simulink library "indi_lib"  (R2018b)
settings: Solver=VariableStepAuto  StartTime=0.0  StopTime=10.0  RelTol=1e-3
values from neighbouring files (symbols this model uses):
  G10 = [          inv_I_b * cross( pos, c_XYZ );          c_XYZ / ceb.m      ]    [indiCeFlapFix.m]    (also in indiCePropFix.m = [          2 * inv_I_b * (cep.k*L + cep.d*M .* repmat(cep.a,)
  G20 = 1 / T_s *      [          inv_I_b * cep.ip * M .* repmat(cep.a,3,1);          zeros( 1, num_motors )      ]    [indiCePropFix.m]
undefined symbols (not defined in the file or in its folder): ap, ca, ceb, cep, indiCePropAffineCntrl, lindi, mtc, sflt, sflt_omega, ts
libraries: filters_lib x6, $bdroot x2, ca_lib x2, ndi_lib x2, simulink x1
settings Model: Creator=Ybeyer  LastModifiedBy=jonas
settings DebuggingCC: LibraryContextMissingDiagnostic=none
settings SFSimCC: SimUseLocalCustomCode=off
settings RTWCC: RTWUseLocalCustomCode=off
settings CodeAppCC: StateflowObjectComments=on

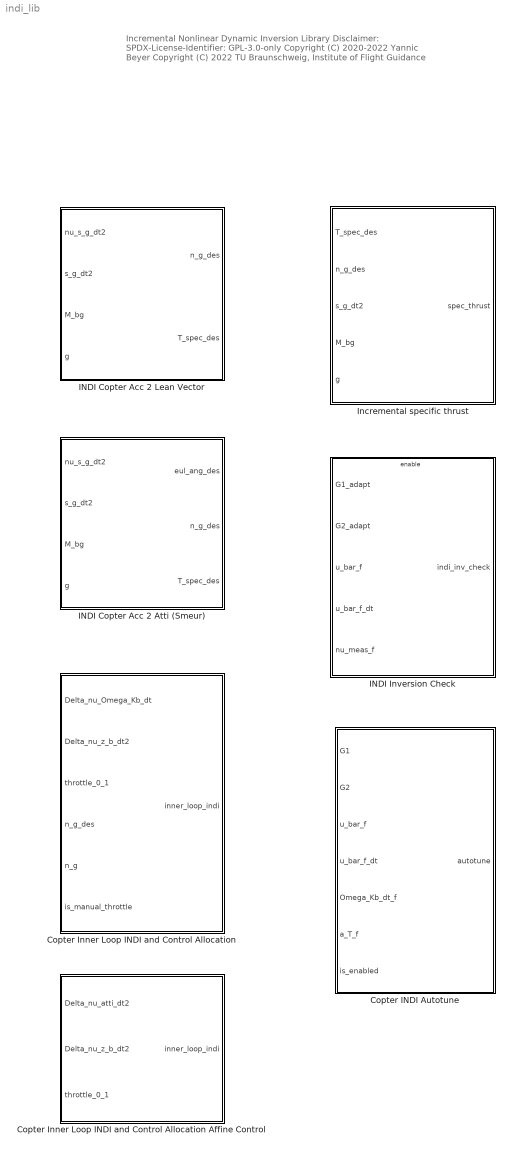
== system indi_lib ==
  note: Incremental Nonlinear Dynamic Inversion Library
      |
      | Disclaimer:
      | SPDX-License-Identifier: GPL-3.0-only
      |
      | Copyright (C) 2020-2022 Yannic Beyer
      | Copyright (C) 2022 TU Braunschweig, Institute of Flight Guidance
  Copter INDI Autotune : Subsystem  mask{rm_atc=lindi.atc.rm, mtc=lindi.mtc, sflt_omega=lindi.sflt.omega, ts=lindi.ts}
      mask prompts: rm_atc "Attitude reference model parameters struct"; mtc "Motor time constant, s"; sflt_omega "Sensor filter cutoff frequency, rad/s"; ts "Sample time, s"
      mask DialogControl DescGroupVar Prompt: Copter INDI Autotune
      mask DialogControl DescTextVar Prompt: This adaptive INDI block is based on: Smeur, E. J., Chu, Q., & De Croon, G. C. (2016). Adaptive incremental nonlinear dynamic inversion for attitude control of micro air vehicles. Journal of Guidance, Control, and Dynamics, 39(3), 450-461.
      mask DialogControl Control2 Prompt: Instead of finding all entries in the G1 and G2 matrix, the number of estimated parameters is 5: one for each: roll, pitch, yaw, vertical acc. (G1) and one for yaw due to propeller acceleration (G2).
  Copter Inner Loop INDI and Control Allocation : Subsystem  mask{cep=ap.cep, ceb=ap.ceb, ca=ap.ca, mtc=ap.mtc, sflt=ap.sflt, ts=ap.ts, is_ce_extern=off}
      mask prompts: cep "Parameters for motor-propeller control effectiveness, see indiCeProp_params_default"; ceb "Parameters for body control effectiveness, see indiCeBody_params_default"; ca "Control allocation parameters, see controlAllocationWlsLoadParams"; mtc "Motor time constant, s"; sflt "Sensor filter parameters, see indiSensFiltLoadParams"; ts "Sample time, s"; is_ce_extern "Enable external control effectiveness"
      mask init:
      | caIndiCopterBlockInit(is_ce_extern);
      mask DialogControl DescGroupVar Prompt: Copter Inner Loop INDI and Control Allocation
  Copter Inner Loop INDI and Control Allocation Affine Control : Subsystem  mask{cep=cep, ceb=ceb, ca=ca, mtc=mtc, sflt=sflt, ts=ts}
      mask prompts: cep "Parameters for motor-propeller control effectiveness, see indiCeProp_params_default"; ceb "Parameters for body control effectiveness, see indiCeBody_params_default"; ca "Control allocation parameters, see controlAllocationWlsLoadParams"; mtc "Motor time constant, s"; sflt "Sensor filter parameters, see indiSensFiltLoadParams"; ts "Sample time, s"
      mask init:
      | u_min = ca.u_min;
      | u_max = ca.u_max;
      | u_d = ca.u_d;
      | 
      | U_min = indiCePropAffineCntrl( cep, ca.u_min );
      | U_max = indiCePropAffineCntrl( cep, ca.u_max );
      | U_d = indiCePropAffineCntrl( cep, ca.u_d );
      | 
      | ca.u_min = U_min;
      | ca.u_max = U_max;
      | ca.u_d = U_d;
      mask DialogControl DescGroupVar Prompt: Copter Inner Loop INDI and Control Allocation with Affine Control
      mask DialogControl DescTextVar Prompt: The special feature of this implementation is that the control effectiveness matrix G1 (or renamed G1U here) remains constant, so it does not need to be scheduled. For this purpose, an artificial control input (here called 0 <= U <= 1) was defined, on which the thrust and the torque depend linearly. The actual control input (duty cycle 0 <= u <= 1) is then calculated non-linearly from the artificial control input U.
  INDI Copter Acc 2 Atti (Smeur) : MATLAB Function  TreatAsAtomicUnit=on
  INDI Copter Acc 2 Lean Vector : MATLAB Function  TreatAsAtomicUnit=on
  INDI Inversion Check : Subsystem  mask{omega_filt=2/(2/sflt_omega + mtc), mask_expr_handling_config=default}
      mask prompts: omega_filt "Filter cutoff frequency (sensor and actuator), rad/s"
      mask init:
      | maskExprHandling(gcbh, mask_expr_handling_config);
      mask TypeOptions mask_expr_handling_config: default | passthrough (tunable)
      mask DialogControl DescGroupVar Prompt: INDI Inversion Check
      mask DialogControl DescTextVar Prompt: Check how good an INDI inversion is. Therefore, the expected and measure pseudo-control signal can be compared.
      mask DialogControl CodeGenerationSettings Prompt: Code Generation Settings
      mask DialogControl maskExprHandlingText Prompt: Mask expression handling
      mask DialogControl maskExprHandlingReadme Prompt: README
      mask DialogControl maskExprHandlingReadme Tooltip: https://github.com/iff-gsc/m-Utils/tree/main/simulink/mask_expression_handling/README.md
      mask DialogControl maskExprHandlingReadme Callback: web('https://github.com/iff-gsc/m-Utils/tree/main/simulink/mask_expression_handling/README.md','-browser')
  Incremental specific thrust : Subsystem  mask{leanfreq=10, leandamp=1, is_enable_checked=off, states_when_enabling=held}
      mask prompts: leanfreq "Natural frequency of attitude reference model, rad/s"; leandamp "Damping ratio of attitude reference model"; is_enable_checked "Activate "Enabled Subsystem""; states_when_enabling "States when enabling:"
      mask init:
      | cntrlBlockInit(is_enable_checked,states_when_enabling);
      mask TypeOptions states_when_enabling: held | reset
      mask DialogControl DescGroupVar Prompt: Incremental specific thrust

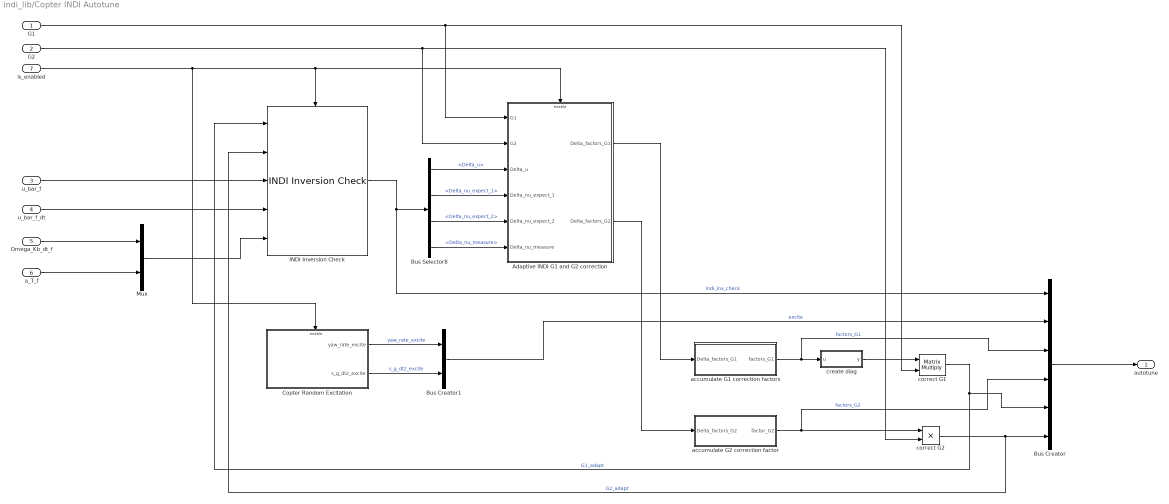
== system indi_lib/Copter INDI Autotune ==
  G1 : Inport
  G2 : Inport  Port=2
  u_bar_f : Inport  Port=3
  u_bar_f_dt : Inport  Port=4
  Omega_Kb_dt_f : Inport  Port=5
  a_T_f : Inport  Port=6
  is_enabled : Inport  Port=7
  Adaptive INDI G1 and G2 correction : Subsystem
  Bus Creator : BusCreator  Inputs=6
  Bus Creator1 : BusCreator  Inputs=2
  Bus Selector8 : BusSelector  OutputSignals=Delta_u,Delta_nu_expect_1,Delta_nu_expect_2,Delta_nu_measure
  Copter Random Excitation : Subsystem
  INDI Inversion Check : $bdroot/INDI Inversion Check  omega_filt=2/(2/sflt_omega + mtc)  mask_expr_handling_config=passthrough (tunable)
  Mux : Mux  Inputs=2
  accumulate G1 correction factors : Subsystem
  accumulate G2 correction factor : Subsystem
  correct G1 : Product  Multiplication=Matrix(*)
  correct G2 : Product
  create diag : MATLAB Function  TreatAsAtomicUnit=on
  autotune : Outport
  wires:
  G1/1 -> Adaptive INDI G1 and G2 correction/1(G1), correct G1/2
  G2/1 -> correct G2/2, Adaptive INDI G1 and G2 correction/2(G2)
  Adaptive INDI G1 and G2 correction/1(Delta_factors_G1) -> accumulate G1 correction factors/1(Delta_factors_G1)
  accumulate G1 correction factors/1(factors_G1) -> Bus Creator/3, create diag/1(u)  "factors_G1"
  accumulate G2 correction factor/1(factor_G2) -> Bus Creator/4, correct G2/1  "factors_G2"
  Adaptive INDI G1 and G2 correction/2(Delta_factors_G2) -> accumulate G2 correction factor/1(Delta_factors_G2)
  Copter Random Excitation/2(s_g_dt2_excite) -> Bus Creator1/2  "s_g_dt2_excite"
  Bus Selector8/2 -> Adaptive INDI G1 and G2 correction/4(Delta_nu_expect_1)  "<Delta_nu_expect_1>"
  Copter Random Excitation/1(yaw_rate_excite) -> Bus Creator1/1  "yaw_rate_excite"
  Bus Selector8/1 -> Adaptive INDI G1 and G2 correction/3(Delta_u)  "<Delta_u>"
  Bus Selector8/3 -> Adaptive INDI G1 and G2 correction/5(Delta_nu_expect_2)  "<Delta_nu_expect_2>"
  INDI Inversion Check/1 -> Bus Creator/1, Bus Selector8/1  "indi_inv_check"
  Bus Selector8/4 -> Adaptive INDI G1 and G2 correction/6(Delta_nu_measure)  "<Delta_nu_measure>"
  Bus Creator1/1 -> Bus Creator/2  "excite"
  Bus Creator/1 -> autotune/1
  Mux/1 -> INDI Inversion Check/5
  u_bar_f/1 -> INDI Inversion Check/3
  u_bar_f_dt/1 -> INDI Inversion Check/4
  Omega_Kb_dt_f/1 -> Mux/1
  a_T_f/1 -> Mux/2
  correct G2/1 -> Bus Creator/6, INDI Inversion Check/2  "G2_adapt"
  correct G1/1 -> INDI Inversion Check/1, Bus Creator/5  "G1_adapt"
  create diag/1(y) -> correct G1/1
  is_enabled/1 -> INDI Inversion Check/Enable, Adaptive INDI G1 and G2 correction/Enable, Copter Random Excitation/Enable

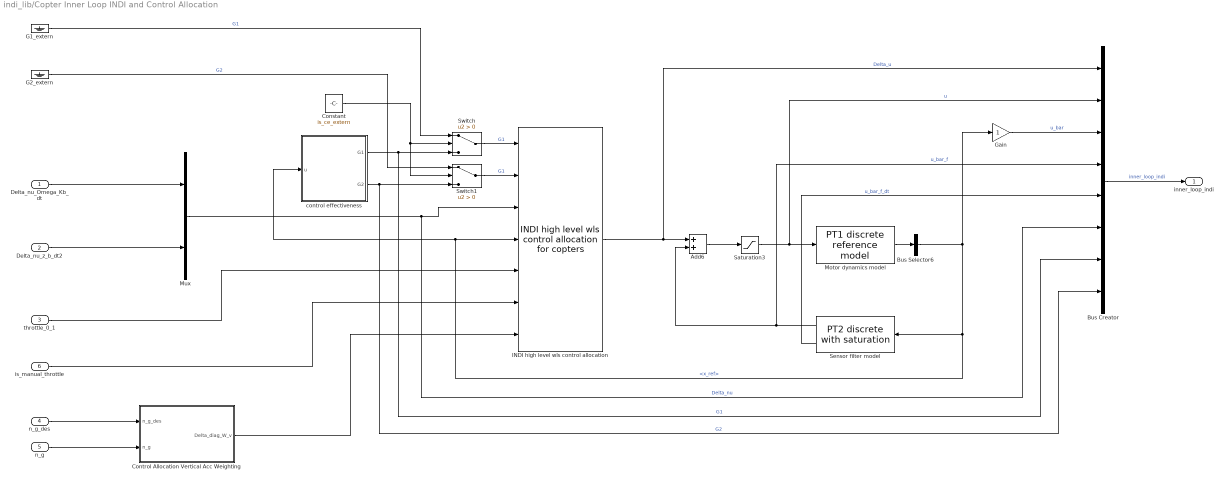
== system indi_lib/Copter Inner Loop INDI and Control Allocation ==
  Delta_nu_Omega_Kb_dt : Inport
  Delta_nu_z_b_dt2 : Inport  Port=2
  throttle_0_1 : Inport  Port=3
  n_g_des : Inport  Port=4
  n_g : Inport  Port=5
  is_manual_throttle : Inport  Port=6
  Add6 : Sum
  Bus Creator : BusCreator  Inputs=8
  Bus Selector6 : BusSelector  OutputSignals=x_ref
  Constant : Constant  Value=is_ce_extern
  Control Allocation Vertical Acc Weighting : MATLAB Function  TreatAsAtomicUnit=on
  G1_extern : Ground
  G2_extern : Ground
  Gain : Gain
  INDI high level wls control allocation : ca_lib/INDI high level wls control allocation for copters  ca=ca  is_Delta_W_v_check=on  is_W_check=off  is_iter_check=off
      settings: SourceProductName=LADAC
  Motor dynamics model : ndi_lib/PT1 discrete reference model  T=mtc  x_max=inf  x_min=-inf  x_dt_max=inf  x_dt_min=-inf  x_init=0
      settings: SourceProductName=LADAC
  Mux : Mux  Inputs=2
  Saturation3 : Saturate  UpperLimit=ca.u_max  LowerLimit=ca.u_min
  Sensor filter model : filters_lib/PT2 discrete with saturation  param_src=internal  omega=sflt.omega  d=sflt.D  x_max=inf  x_min=-inf  x_dt_max=inf  x_dt_min=-inf  x_dt2_max=inf  x_dt2_min=-inf  y_0_src=internal  x_init=0  y_dt_0_src=internal  x_dt_init=0  is_y_dt_checked=on  is_y_dt2_checked=off  is_external_reset_checked=off  mask_expr_handling_config=default
      settings: SourceProductName=LADAC
  Switch : Switch  Criteria=u2 > Threshold
  Switch1 : Switch  Criteria=u2 > Threshold
  control effectiveness : Subsystem  mask{cep=cep, ceb=ceb, ts=ts, u_min=ca.u_min}
      mask prompts: cep "propeller control effectiveness struct, see cntrlEffectPropLoadParams"; ceb "body control effectiveness struct, see cntrlEffectBodyLoadParams"; ts "controller sample time, s"
      mask init:
      | [G10,G20] = indiCePropFix( cep, ceb, ts );
  inner_loop_indi : Outport
  wires:
  is_manual_throttle/1 -> INDI high level wls control allocation/6
  n_g/1 -> Control Allocation Vertical Acc Weighting/2(n_g)
  n_g_des/1 -> Control Allocation Vertical Acc Weighting/1(n_g_des)
  Control Allocation Vertical Acc Weighting/1(Delta_diag_W_v) -> INDI high level wls control allocation/7
  Bus Creator/1 -> inner_loop_indi/1  "inner_loop_indi"
  Gain/1 -> Bus Creator/3  "u_bar"
  Delta_nu_z_b_dt2/1 -> Mux/2
  control effectiveness/2(G2) -> Switch1/3, Bus Creator/8  "G2"
  Delta_nu_Omega_Kb_dt/1 -> Mux/1
  Add6/1 -> Saturation3/1
  Motor dynamics model/1 -> Bus Selector6/1
  control effectiveness/1(G1) -> Bus Creator/7, Switch/3  "G1"
  Bus Selector6/1 -> control effectiveness/1(u), INDI high level wls control allocation/4, Sensor filter model/1, Gain/1  "<x_ref>"
  throttle_0_1/1 -> INDI high level wls control allocation/5
  INDI high level wls control allocation/1 -> Add6/1, Bus Creator/1  "Delta_u"
  Saturation3/1 -> Motor dynamics model/1, Bus Creator/2  "u"
  Mux/1 -> Bus Creator/6, INDI high level wls control allocation/3  "Delta_nu"
  Sensor filter model/1 -> Add6/2, Bus Creator/4  "u_bar_f"
  Switch/1 -> INDI high level wls control allocation/1  "G1"
  Switch1/1 -> INDI high level wls control allocation/2  "G1"
  G1_extern/1 -> Switch/1  "G1"
  G2_extern/1 -> Switch1/1  "G2"
  Constant/1 -> Switch1/2, Switch/2
  Sensor filter model/2 -> Bus Creator/5  "u_bar_f_dt"

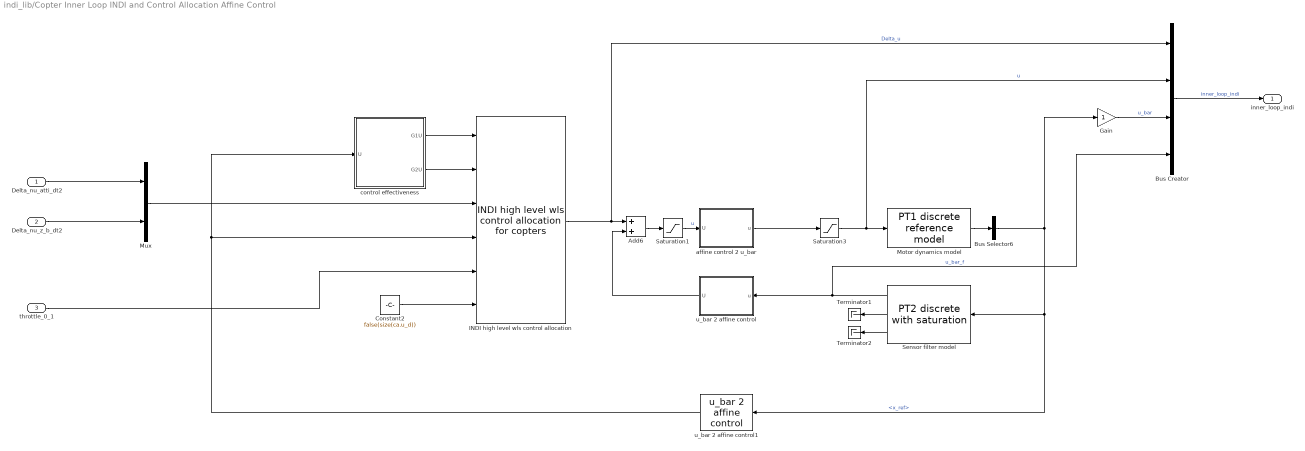
== system indi_lib/Copter Inner Loop INDI and Control Allocation Affine Control ==
  Delta_nu_atti_dt2 : Inport
  Delta_nu_z_b_dt2 : Inport  Port=2
  throttle_0_1 : Inport  Port=3
  Add6 : Sum
  Bus Creator : BusCreator  Inputs=4
  Bus Selector6 : BusSelector  OutputSignals=x_ref
  Constant2 : Constant  Value=false(size(ca.u_d))
  Gain : Gain
  INDI high level wls control allocation : ca_lib/INDI high level wls control allocation for copters  ca=ca  is_Delta_W_v_check=off  is_W_check=off  is_iter_check=off
      settings: SourceProductName=LADAC
  Motor dynamics model : ndi_lib/PT1 discrete reference model  T=mtc  x_max=inf  x_min=-inf  x_dt_max=inf  x_dt_min=-inf  x_init=0
      settings: SourceProductName=LADAC
  Mux : Mux  Inputs=2
  Saturation1 : Saturate  UpperLimit=indiCePropAffineCntrl( cep, ca.u_max )  LowerLimit=indiCePropAffineCntrl( cep, ca.u_min )
  Saturation3 : Saturate  UpperLimit=u_max  LowerLimit=u_min
  Sensor filter model : filters_lib/PT2 discrete with saturation  param_src=internal  omega=sflt.omega  d=sflt.D  x_dt2_max=inf  x_dt2_min=-inf  x_dt_max=inf  x_dt_min=-inf  x_max=inf  x_min=-inf  y_0_src=internal  x_init=0  y_dt_0_src=internal  x_dt_init=0  is_y_dt_checked=on  is_y_dt2_checked=on
      settings: SourceProductName=LADAC
  Terminator1 : Terminator
  Terminator2 : Terminator
  affine control 2 u_bar : Subsystem  mask{cep=cep}
  control effectiveness : Subsystem  mask{cep=cep, ceb=ceb, ts=ts, u_min=ca.u_min}
      mask prompts: cep "propeller control effectiveness struct, see cntrlEffectPropLoadParams"; ceb "body control effectiveness struct, see cntrlEffectBodyLoadParams"; ts "controller sample time, s"
      mask init:
      | [G10,G20] = indiCePropFix( cep, ceb, ts );
      | 
      | u_max = ones(4,1);
      | 
      | omega_max = motorStaticSpeed( cep.kt, cep.ri, cep.vb, cep.d, u_max );
      | omega2 = diag( omega_max.^2 );
      | 
      | G1U = 0.5 * G10 * omega2;
  u_bar 2 affine control : Subsystem  mask{cep=cep}
  u_bar 2 affine control1 : $bdroot/Copter Inner Loop INDI and Control Allocation Affine Control/u_bar 2 affine control  cep=cep
  inner_loop_indi : Outport
  wires:
  throttle_0_1/1 -> INDI high level wls control allocation/5
  Sensor filter model/1 -> Bus Creator/4, u_bar 2 affine control/1(u)  "u_bar_f"
  Sensor filter model/2 -> Terminator1/1
  Add6/1 -> Saturation1/1
  INDI high level wls control allocation/1 -> Bus Creator/1, Add6/1  "Delta_u"
  affine control 2 u_bar/1(u) -> Saturation3/1
  Motor dynamics model/1 -> Bus Selector6/1
  Constant2/1 -> INDI high level wls control allocation/6
  Sensor filter model/3 -> Terminator2/1
  Delta_nu_atti_dt2/1 -> Mux/1
  Saturation3/1 -> Bus Creator/2, Motor dynamics model/1  "u"
  u_bar 2 affine control1/1 -> control effectiveness/1(U), INDI high level wls control allocation/4
  Bus Selector6/1 -> Gain/1, u_bar 2 affine control1/1, Sensor filter model/1  "<x_ref>"
  Delta_nu_z_b_dt2/1 -> Mux/2
  Saturation1/1 -> affine control 2 u_bar/1(U)  "u"
  Mux/1 -> INDI high level wls control allocation/3
  u_bar 2 affine control/1(U) -> Add6/2
  control effectiveness/1(G1U) -> INDI high level wls control allocation/1
  control effectiveness/2(G2U) -> INDI high level wls control allocation/2
  Bus Creator/1 -> inner_loop_indi/1  "inner_loop_indi"
  Gain/1 -> Bus Creator/3  "u_bar"

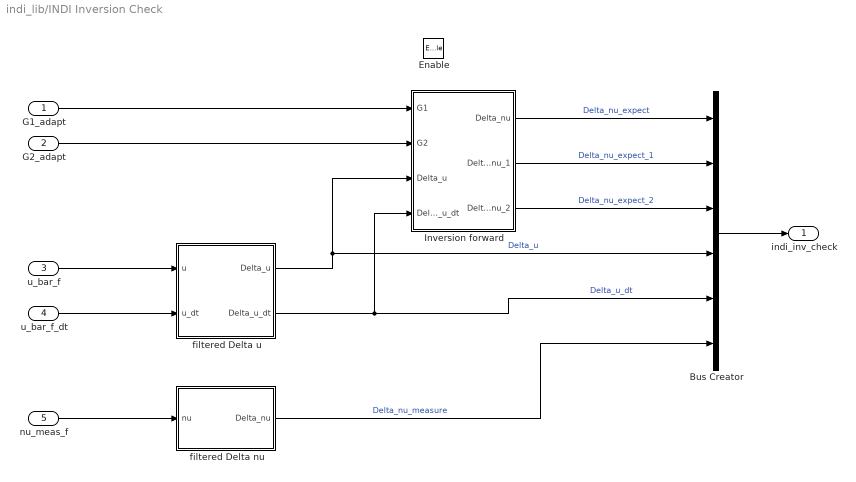
== system indi_lib/INDI Inversion Check ==
  G1_adapt : Inport
  G2_adapt : Inport  Port=2
  u_bar_f : Inport  Port=3
  u_bar_f_dt : Inport  Port=4
  nu_meas_f : Inport  Port=5
  Enable : EnablePort
  Bus Creator : BusCreator  Inputs=6
  Inversion forward : Subsystem
  filtered Delta nu : Subsystem
  filtered Delta u : Subsystem
  indi_inv_check : Outport
  wires:
  Inversion forward/3(Delta_nu_2) -> Bus Creator/3  "Delta_nu_expect_2"
  Inversion forward/2(Delta_nu_1) -> Bus Creator/2  "Delta_nu_expect_1"
  G1_adapt/1 -> Inversion forward/1(G1)
  G2_adapt/1 -> Inversion forward/2(G2)
  Inversion forward/1(Delta_nu) -> Bus Creator/1  "Delta_nu_expect"
  u_bar_f/1 -> filtered Delta u/1(u)
  filtered Delta u/1(Delta_u) -> Inversion forward/3(Delta_u), Bus Creator/4  "Delta_u"
  filtered Delta nu/1(Delta_nu) -> Bus Creator/6  "Delta_nu_measure"
  nu_meas_f/1 -> filtered Delta nu/1(nu)
  u_bar_f_dt/1 -> filtered Delta u/2(u_dt)
  filtered Delta u/2(Delta_u_dt) -> Bus Creator/5, Inversion forward/4(Delta_u_dt)  "Delta_u_dt"
  Bus Creator/1 -> indi_inv_check/1

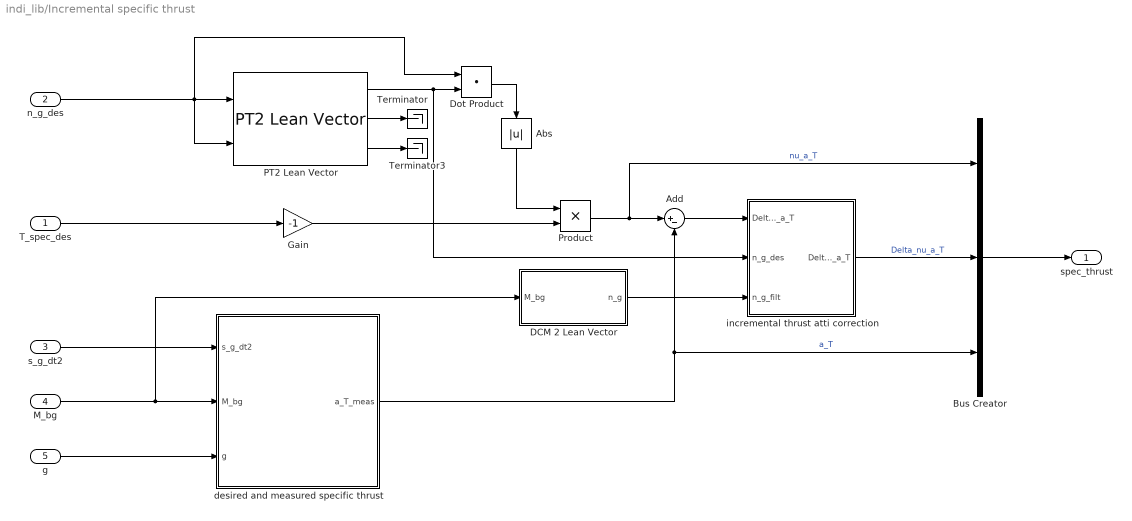
== system indi_lib/Incremental specific thrust ==
  T_spec_des : Inport
  n_g_des : Inport  Port=2
  s_g_dt2 : Inport  Port=3
  M_bg : Inport  Port=4
  g : Inport  Port=5
  Abs : Abs
  Add : Sum  Inputs=|+-
  Bus Creator : BusCreator  Inputs=3
  DCM 2 Lean Vector : MATLAB Function  TreatAsAtomicUnit=on
  Dot Product : DotProduct  InputSameDT=on  OutDataTypeStr=Inherit: Inherit via internal rule
  Gain : Gain  Gain=-1
  PT2 Lean Vector : filters_lib/PT2 Lean Vector  omega=leanfreq  d=leandamp  x_dt2_max=inf  x_dt2_min=-inf  x_dt_max=inf  x_dt_min=-inf  x_max=inf  x_min=-inf  x_init=0  x_dt_init=0
      settings: SourceProductName=LADAC
  Product : Product
  Terminator : Terminator
  Terminator3 : Terminator
  desired and measured specific thrust : MATLAB Function  TreatAsAtomicUnit=on
  incremental thrust atti correction : MATLAB Function  TreatAsAtomicUnit=on
  spec_thrust : Outport
  wires:
  T_spec_des/1 -> Gain/1
  desired and measured specific thrust/1(a_T_meas) -> Add/2, Bus Creator/3  "a_T"
  Add/1 -> incremental thrust atti correction/1("Delta_nu_a_T ")
  s_g_dt2/1 -> desired and measured specific thrust/1(s_g_dt2)
  M_bg/1 -> DCM 2 Lean Vector/1(M_bg), desired and measured specific thrust/2(M_bg)
  g/1 -> desired and measured specific thrust/3(g)
  Gain/1 -> Product/2
  n_g_des/1 -> Dot Product/1, PT2 Lean Vector/2, PT2 Lean Vector/1
  PT2 Lean Vector/1 -> incremental thrust atti correction/2(n_g_des), Dot Product/2
  PT2 Lean Vector/2 -> Terminator/1
  PT2 Lean Vector/3 -> Terminator3/1
  Dot Product/1 -> Abs/1
  Product/1 -> Bus Creator/1, Add/1  "nu_a_T"
  Abs/1 -> Product/1
  incremental thrust atti correction/1(Delta_nu_a_T) -> Bus Creator/2  "Delta_nu_a_T"
  DCM 2 Lean Vector/1(n_g) -> incremental thrust atti correction/3(n_g_filt)
  Bus Creator/1 -> spec_thrust/1

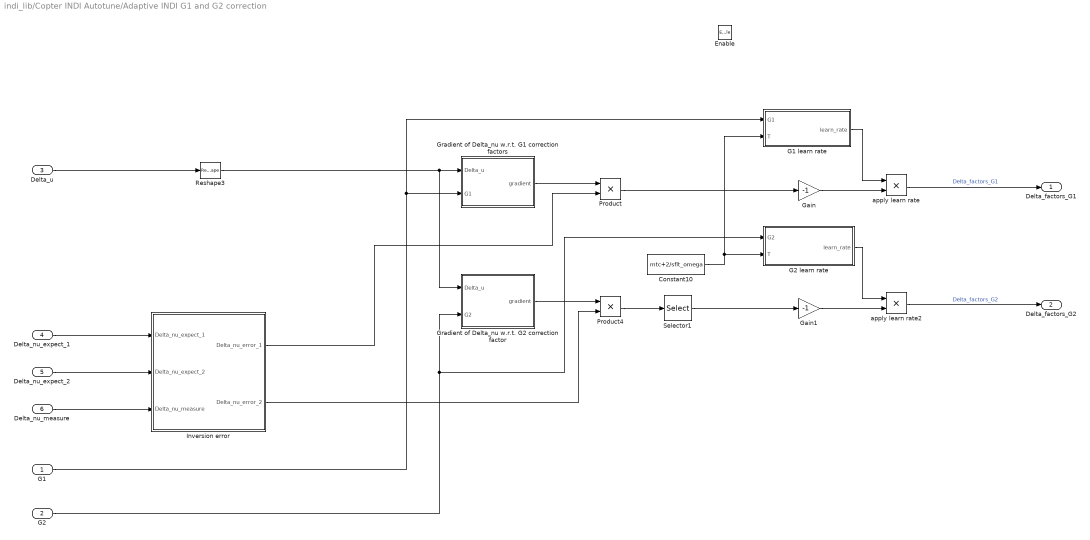
== system indi_lib/Copter INDI Autotune/Adaptive INDI G1 and G2 correction ==
  G1 : Inport
  G2 : Inport  Port=2
  Delta_u : Inport  Port=3
  Delta_nu_expect_1 : Inport  Port=4
  Delta_nu_expect_2 : Inport  Port=5
  Delta_nu_measure : Inport  Port=6
  Enable : EnablePort
  Constant10 : Constant  Value=mtc+2/sflt_omega
  G1 learn rate : MATLAB Function  TreatAsAtomicUnit=on
  G2 learn rate : MATLAB Function  TreatAsAtomicUnit=on
  Gain : Gain  Gain=-1
  Gain1 : Gain  Gain=-1
  Gradient of Delta_nu w.r.t. G1 correction factors : Subsystem
  Gradient of Delta_nu w.r.t. G2 correction factor : Subsystem
  Inversion error : Subsystem
  Product : Product
  Product4 : Product
  Reshape3 : Reshape  OutputDimensionality=Column vector (2-D)
  Selector1 : Selector  InputPortWidth=4  IndexOptions=Index vector (dialog)  Indices=3  OutputSizes=1
  apply learn rate : Product
  apply learn rate2 : Product
  Delta_factors_G1 : Outport  OutputWhenDisabled=reset  InitialOutput=0
  Delta_factors_G2 : Outport  Port=2  OutputWhenDisabled=reset  InitialOutput=0
  wires:
  Reshape3/1 -> Gradient of Delta_nu w.r.t. G1 correction factors/1(Delta_u), Gradient of Delta_nu w.r.t. G2 correction factor/1(Delta_u)
  Delta_u/1 -> Reshape3/1
  Product/1 -> Gain/1
  Inversion error/1(Delta_nu_error_1) -> Product/2
  Product4/1 -> Selector1/1
  Selector1/1 -> Gain1/1
  apply learn rate/1 -> Delta_factors_G1/1  "Delta_factors_G1"
  apply learn rate2/1 -> Delta_factors_G2/1  "Delta_factors_G2"
  Gain1/1 -> apply learn rate2/2
  Gain/1 -> apply learn rate/2
  Gradient of Delta_nu w.r.t. G2 correction factor/1(gradient) -> Product4/1
  Gradient of Delta_nu w.r.t. G1 correction factors/1(gradient) -> Product/1
  G2 learn rate/1(learn_rate) -> apply learn rate2/1
  G1/1 -> G1 learn rate/1(G1), Gradient of Delta_nu w.r.t. G1 correction factors/2(G1)
  G2/1 -> G2 learn rate/1(G2), Gradient of Delta_nu w.r.t. G2 correction factor/2(G2)
  G1 learn rate/1(learn_rate) -> apply learn rate/1
  Inversion error/2(Delta_nu_error_2) -> Product4/2
  Constant10/1 -> G2 learn rate/2(T), G1 learn rate/2(T)
  Delta_nu_expect_1/1 -> Inversion error/1(Delta_nu_expect_1)
  Delta_nu_expect_2/1 -> Inversion error/2(Delta_nu_expect_2)
  Delta_nu_measure/1 -> Inversion error/3(Delta_nu_measure)

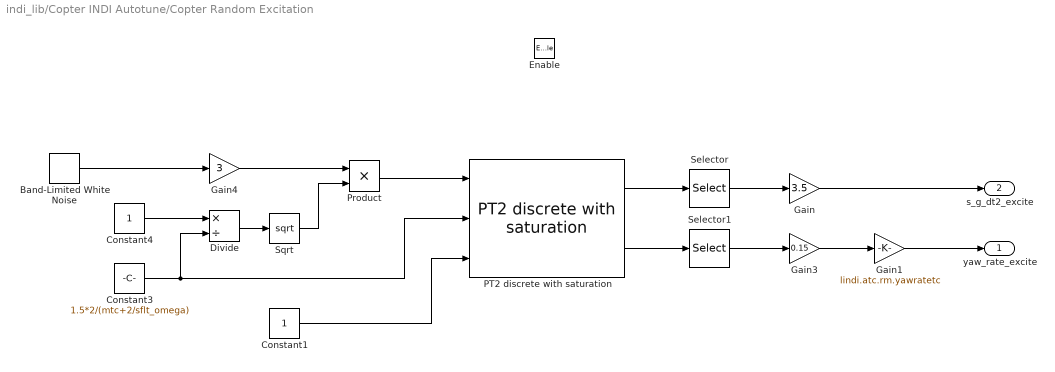
== system indi_lib/Copter INDI Autotune/Copter Random Excitation ==
  Enable : EnablePort  StatesWhenEnabling=reset
  Band-Limited White Noise : simulink/Sources/Band-Limited White Noise  Cov=[0.025]  Ts=ts  seed=[23341,23342,23343,23344]
  Constant1 : Constant
  Constant3 : Constant  Value=1.5*2/(mtc+2/sflt_omega)
  Constant4 : Constant
  Divide : Product  Inputs=*/
  Gain : Gain  Gain=3.5
  Gain1 : Gain  Gain=lindi.atc.rm.yawratetc
  Gain3 : Gain  Gain=0.15
  Gain4 : Gain  Gain=3
  PT2 discrete with saturation : filters_lib/PT2 discrete with saturation  param_src=external  omega=1  d=1  x_dt2_max=inf  x_dt2_min=-inf  x_dt_max=inf  x_dt_min=-inf  x_max=inf  x_min=-inf  y_0_src=internal  x_init=0  y_dt_0_src=internal  x_dt_init=0  is_y_dt_checked=on  is_y_dt2_checked=off
      settings: SourceProductName=LADAC
  Product : Product
  Selector : Selector  InputPortWidth=4  IndexOptions=Index vector (dialog)  Indices=1:3  OutputSizes=1
  Selector1 : Selector  InputPortWidth=4  IndexOptions=Index vector (dialog)  Indices=4  OutputSizes=1
  Sqrt : Sqrt  SaturateOnIntegerOverflow=on
  yaw_rate_excite : Outport  OutputWhenDisabled=reset  InitialOutput=0
  s_g_dt2_excite : Outport  Port=2  OutputWhenDisabled=reset  InitialOutput=0
  wires:
  Gain1/1 -> yaw_rate_excite/1
  PT2 discrete with saturation/1 -> Selector/1
  Constant1/1 -> PT2 discrete with saturation/3
  Gain/1 -> s_g_dt2_excite/1
  PT2 discrete with saturation/2 -> Selector1/1
  Sqrt/1 -> Product/2
  Selector/1 -> Gain/1
  Constant4/1 -> Divide/1
  Selector1/1 -> Gain3/1
  Product/1 -> PT2 discrete with saturation/1
  Constant3/1 -> Divide/2, PT2 discrete with saturation/2
  Band-Limited White Noise/1 -> Gain4/1
  Gain3/1 -> Gain1/1
  Gain4/1 -> Product/1
  Divide/1 -> Sqrt/1

== system indi_lib/Copter INDI Autotune/accumulate G1 correction factors ==
  Delta_factors_G1 : Inport
  Add : Sum
  Delay : Delay  DelayLength=1  InitialCondition=1
  Saturation1 : Saturate  UpperLimit=0.1  LowerLimit=-0.1
  Saturation2 : Saturate  UpperLimit=4  LowerLimit=0.25
  factors_G1 : Outport
  wires:
  Delay/1 -> Add/2, factors_G1/1
  Saturation2/1 -> Delay/1
  Saturation1/1 -> Add/1
  Add/1 -> Saturation2/1
  Delta_factors_G1/1 -> Saturation1/1

== system indi_lib/Copter INDI Autotune/accumulate G2 correction factor ==
  Delta_factors_G2 : Inport
  Add1 : Sum
  Delay1 : Delay  DelayLength=1  InitialCondition=1
  Saturation1 : Saturate  UpperLimit=0.1  LowerLimit=-0.1
  Saturation3 : Saturate  UpperLimit=4  LowerLimit=0.25
  factor_G2 : Outport  PortDimensions=1
  wires:
  Saturation3/1 -> Delay1/1
  Saturation1/1 -> Add1/1
  Delta_factors_G2/1 -> Saturation1/1
  Delay1/1 -> Add1/2, factor_G2/1
  Add1/1 -> Saturation3/1

== system indi_lib/Copter Inner Loop INDI and Control Allocation/control effectiveness ==
  u : Inport
  Constant1 : Constant  Value=u_min
  MATLAB Function : MATLAB Function  TreatAsAtomicUnit=on
  Max : MinMax  Function=max  Inputs=2  OutDataTypeStr=Inherit: Inherit via back propagation
  G1 : Outport
  G2 : Outport  Port=2
  wires:
  MATLAB Function/2(G2) -> G2/1
  MATLAB Function/1(G1) -> G1/1
  Max/1 -> MATLAB Function/1(u)
  Constant1/1 -> Max/2
  u/1 -> Max/1

== system indi_lib/Copter Inner Loop INDI and Control Allocation Affine Control/affine control 2 u_bar ==
  U : Inport
  MATLAB Function3 : MATLAB Function  TreatAsAtomicUnit=on
  u : Outport
  wires:
  MATLAB Function3/1(u) -> u/1
  U/1 -> MATLAB Function3/1(U)

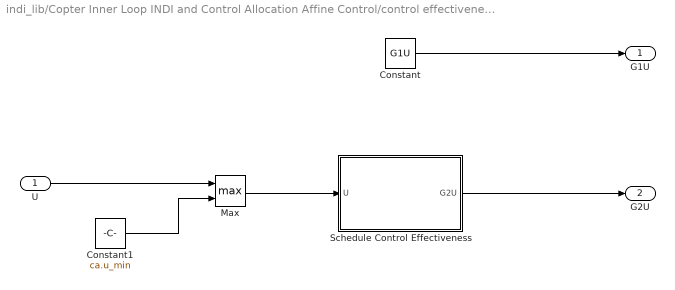
== system indi_lib/Copter Inner Loop INDI and Control Allocation Affine Control/control effectiveness ==
  U : Inport
  Constant : Constant  Value=G1U
  Constant1 : Constant  Value=ca.u_min
  Max : MinMax  Function=max  Inputs=2  OutDataTypeStr=Inherit: Inherit via back propagation
  Schedule Control Effectiveness : MATLAB Function  TreatAsAtomicUnit=on
  G1U : Outport
  G2U : Outport  Port=2
  wires:
  U/1 -> Max/1
  Constant1/1 -> Max/2
  Max/1 -> Schedule Control Effectiveness/1(U)
  Schedule Control Effectiveness/1(G2U) -> G2U/1
  Constant/1 -> G1U/1

== system indi_lib/Copter Inner Loop INDI and Control Allocation Affine Control/u_bar 2 affine control ==
  u : Inport
  indiCePropAffineCntrl : MATLAB Function  TreatAsAtomicUnit=on
  U : Outport
  wires:
  u/1 -> indiCePropAffineCntrl/1(u)
  indiCePropAffineCntrl/1(U) -> U/1

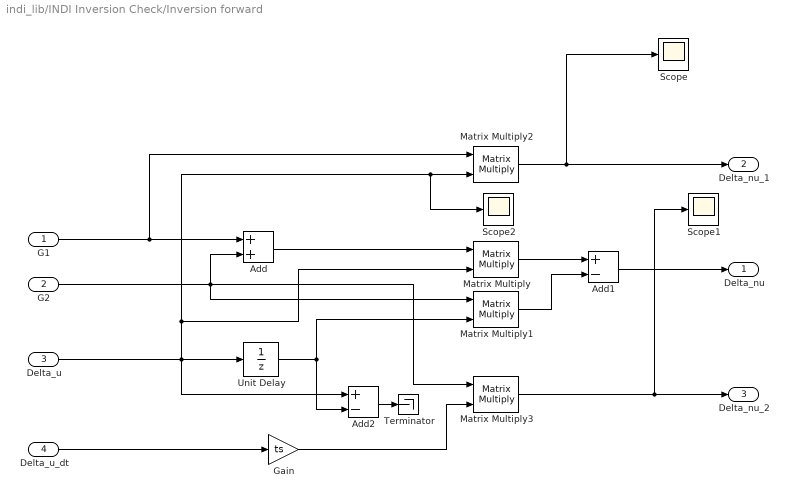
== system indi_lib/INDI Inversion Check/Inversion forward ==
  G1 : Inport
  G2 : Inport  Port=2
  Delta_u : Inport  Port=3
  Delta_u_dt : Inport  Port=4
  Add : Sum
  Add1 : Sum  Inputs=+-
  Add2 : Sum  Inputs=+-
  Gain : Gain  Gain=ts
  Matrix Multiply{,1..3} (4 alike) : Product  Multiplication=Matrix(*)
  Scope : Scope
  Scope1 : Scope
  Scope2 : Scope
  Terminator : Terminator
  Unit Delay : UnitDelay  SampleTime=-1
  Delta_nu : Outport
  Delta_nu_1 : Outport  Port=2
  Delta_nu_2 : Outport  Port=3
  wires:
  Add2/1 -> Terminator/1
  Gain/1 -> Matrix Multiply3/2
  Matrix Multiply3/1 -> Delta_nu_2/1, Scope1/1
  Delta_u_dt/1 -> Gain/1
  Matrix Multiply2/1 -> Delta_nu_1/1, Scope/1
  Matrix Multiply1/1 -> Add1/2
  Add1/1 -> Delta_nu/1
  Add/1 -> Matrix Multiply/1
  Unit Delay/1 -> Matrix Multiply1/2, Add2/2
  Matrix Multiply/1 -> Add1/1
  G2/1 -> Add/2, Matrix Multiply1/1, Matrix Multiply3/1
  Delta_u/1 -> Add2/1, Unit Delay/1, Matrix Multiply/2, Matrix Multiply2/2, Scope2/1
  G1/1 -> Matrix Multiply2/1, Add/1

== system indi_lib/INDI Inversion Check/filtered Delta nu ==
  nu : Inport
  Add2 : Sum  Inputs=+-
  PT2 discrete with saturation1 : filters_lib/PT2 discrete with saturation  param_src=internal  omega=omega_filt  d=1  x_max=inf  x_min=-inf  x_dt_max=inf  x_dt_min=-inf  x_dt2_max=inf  x_dt2_min=-inf  y_0_src=external  x_init=0  y_dt_0_src=internal  x_dt_init=0  is_y_dt_checked=off  is_y_dt2_checked=off  is_external_reset_checked=off
      settings: SourceProductName=LADAC
  Delta_nu : Outport
  wires:
  PT2 discrete with saturation1/1 -> Add2/2
  Add2/1 -> Delta_nu/1  "Delta_nu_measure"
  nu/1 -> Add2/1, PT2 discrete with saturation1/1, PT2 discrete with saturation1/2

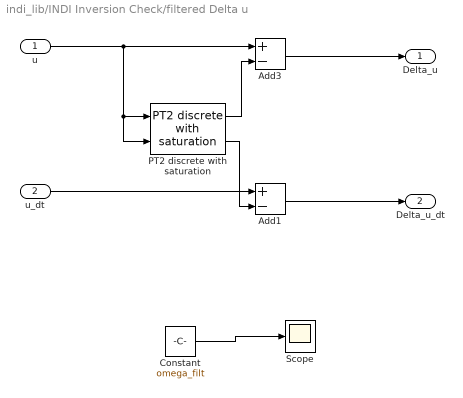
== system indi_lib/INDI Inversion Check/filtered Delta u ==
  u : Inport
  u_dt : Inport  Port=2
  Add1 : Sum  Inputs=+-
  Add3 : Sum  Inputs=+-
  Constant : Constant  Value=omega_filt
  PT2 discrete with saturation : filters_lib/PT2 discrete with saturation  param_src=internal  omega=omega_filt  d=1  x_max=inf  x_min=-inf  x_dt_max=inf  x_dt_min=-inf  x_dt2_max=inf  x_dt2_min=-inf  y_0_src=external  x_init=0  y_dt_0_src=internal  x_dt_init=0  is_y_dt_checked=on  is_y_dt2_checked=off  is_external_reset_checked=off
      settings: SourceProductName=LADAC
  Scope : Scope
  Delta_u : Outport
  Delta_u_dt : Outport  Port=2
  wires:
  Constant/1 -> Scope/1
  PT2 discrete with saturation/1 -> Add3/2
  u/1 -> Add3/1, PT2 discrete with saturation/1, PT2 discrete with saturation/2
  Add3/1 -> Delta_u/1
  PT2 discrete with saturation/2 -> Add1/2
  u_dt/1 -> Add1/1
  Add1/1 -> Delta_u_dt/1

== system indi_lib/Copter INDI Autotune/Adaptive INDI G1 and G2 correction/Gradient of Delta_nu w.r.t. G1 correction factors ==
  Delta_u : Inport
  G1 : Inport  Port=2
  Matrix Multiply5 : Product  Multiplication=Matrix(*)
  gradient : Outport
  wires:
  G1/1 -> Matrix Multiply5/1
  Matrix Multiply5/1 -> gradient/1
  Delta_u/1 -> Matrix Multiply5/2

== system indi_lib/Copter INDI Autotune/Adaptive INDI G1 and G2 correction/Gradient of Delta_nu w.r.t. G2 correction factor ==
  Delta_u : Inport
  G2 : Inport  Port=2
  Add : Sum  Inputs=+-
  Matrix Multiply7 : Product  Multiplication=Matrix(*)
  Unit Delay : UnitDelay  SampleTime=-1
  gradient : Outport
  wires:
  Delta_u/1 -> Unit Delay/1, Add/1
  Matrix Multiply7/1 -> gradient/1
  G2/1 -> Matrix Multiply7/1
  Unit Delay/1 -> Add/2
  Add/1 -> Matrix Multiply7/2

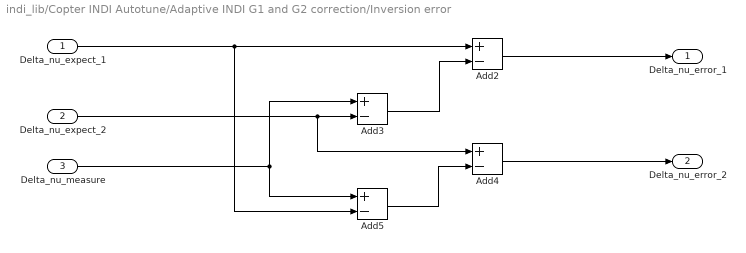
== system indi_lib/Copter INDI Autotune/Adaptive INDI G1 and G2 correction/Inversion error ==
  Delta_nu_expect_1 : Inport
  Delta_nu_expect_2 : Inport  Port=2
  Delta_nu_measure : Inport  Port=3
  Add{2..5} (4 alike) : Sum  Inputs=+-
  Delta_nu_error_1 : Outport
  Delta_nu_error_2 : Outport  Port=2
  wires:
  Add5/1 -> Add4/2
  Add2/1 -> Delta_nu_error_1/1
  Add3/1 -> Add2/2
  Delta_nu_expect_2/1 -> Add3/2, Add4/1
  Add4/1 -> Delta_nu_error_2/1
  Delta_nu_measure/1 -> Add3/1, Add5/1
  Delta_nu_expect_1/1 -> Add5/2, Add2/1

== matlab function indi_lib/INDI Copter Acc 2 Lean Vector ==
  data: nu_s_g_dt2 input; n_g_des output; s_g_dt2 input; M_bg input; g input; T_spec_des output
function [n_g_des,T_spec_des] = indiCopterAcc2LeanVector( nu_s_g_dt2, s_g_dt2, M_bg, g )
[n_g_des,T_spec_des] = indiCopterAcc2LeanVector( nu_s_g_dt2, s_g_dt2, M_bg, g );
end

== matlab function indi_lib/Copter Inner Loop INDI and Control Allocation Affine Control/control effectiveness/Schedule Control Effectiveness ==
  data: G20 parameter; omega_max parameter; U input; G2U output
function G2U = fcn( G20, omega_max, U ) %#codegen

omega_dU = diag( divideFinite( omega_max/2, sqrtReal( U ) ) );

G2U = G20 * omega_dU;

end

== matlab function indi_lib/INDI Copter Acc 2 Atti (Smeur) ==
  data: eul_ang_des output; nu_s_g_dt2 input; n_g_des output; s_g_dt2 input; M_bg input; g input; T_spec_des output
function [eul_ang_des,n_g_des,T_spec_des] = indiCopterAcc2AttiSmeur( nu_s_g_dt2, s_g_dt2, M_bg, g )
[eul_ang_des,T_spec_des,n_g_des] = indiCopterAcc2AttiSmeur( nu_s_g_dt2, s_g_dt2, M_bg, g );
end

== matlab function indi_lib/Incremental specific thrust/incremental thrust atti correction ==
  data: Delta_nu_a_T input; n_g_des input; Delta_nu_a_T output; n_g_filt input
function Delta_nu_a_T = fcn(Delta_nu_a_T,n_g_des,n_g_filt)

proj = dot(n_g_filt,n_g_des);
if proj<0
    Delta_nu_a_T(:) = 0;
else
    Delta_nu_a_T(:) = proj*Delta_nu_a_T;
end

end

== matlab function indi_lib/Incremental specific thrust/DCM 2 Lean Vector ==
  data: M_bg input; n_g output
function n_g = dcm2LeanVector( M_bg )
n_g = dcm2LeanVector( M_bg );
end

== matlab function indi_lib/Copter Inner Loop INDI and Control Allocation/Control Allocation Vertical Acc Weighting ==
  data: n_g_des input; Delta_diag_W_v output; n_g input; ca parameter
function Delta_diag_W_v = caWlsCopterUpset(n_g_des,n_g,ca)
Delta_diag_W_v = caWlsCopterUpset(n_g_des,n_g,ca);
end

== matlab function indi_lib/Copter Inner Loop INDI and Control Allocation/control effectiveness/MATLAB Function ==
  data: cep parameter; G10 parameter; G20 parameter; u input; G1 output; G2 output
function [G1,G2] = indiCePropVar( cep, G10, G20, u ) %#codegen
[G1,G2] = indiCePropVar( cep, G10, G20, u );
end

== matlab function indi_lib/Copter INDI Autotune/Adaptive INDI G1 and G2 correction/G1 learn rate ==
  data: G1 input; learn_rate output; T input; rm_atc parameter
function learn_rate = fcn(G1,T, rm_atc)
learn_rate = zeros(4,1);
G11_mean = mean(abs(G1(1,:)));
G12_mean = mean(abs(G1(2,:)));
G13_mean = mean(abs(G1(3,:)));
G14_mean = mean(abs(G1(4,:)));
learn_rate(1) = 0.02/T / (0.6*2/9.81*rm_atc.leanfreq^2*G11_mean);
learn_rate(2) = 0.02/T / (0.6*2/9.81*rm_atc.leanfreq^2*G12_mean);
learn_rate(3) = 0.0225/T / (10*0.1*rm_atc.yawratemax/rm_atc.yawratetc*G13_mean);
learn_rate(4) = 0.01/T / (0.6*2*G14_mean);
end

== matlab function indi_lib/Copter Inner Loop INDI and Control Allocation Affine Control/u_bar 2 affine control/indiCePropAffineCntrl ==
  data: u input; U output; cep parameter
function U = fcn(u,cep)
U = indiCePropAffineCntrl( cep, u );
end

== matlab function indi_lib/Copter INDI Autotune/Adaptive INDI G1 and G2 correction/G2 learn rate ==
  data: G2 input; learn_rate output; T input; rm_atc parameter; sflt_omega parameter; ts parameter; mtc parameter
function learn_rate = fcn(G2,T, rm_atc, sflt_omega, ts, mtc)
G23_mean = mean(abs(G2(3,:)));
learn_rate =  0.015/T / (10*0.1*rm_atc.yawratemax/rm_atc.yawratetc*1/(2/sflt_omega + mtc)*ts*G23_mean);
end

== matlab function indi_lib/Copter Inner Loop INDI and Control Allocation Affine Control/affine control 2 u_bar/MATLAB Function3 ==
  data: U input; u output; cep parameter
function u = fcn(U,cep)

% u = ((2^(1/2)*(cep.kt*U*(cep.kt^3 - cep.kt*(cep.kt^4 + 4*cep.ri*cep.vb*cep.d*cep.kt)^(1/2) ...
%     + 2*cep.ri*cep.vb*cep.d)).^(1/2) - cep.kt^2).^2 - cep.kt^4)/(4*cep.kt*cep.ri*cep.vb*cep.d);
% u = ((U*((cep.kt^4 + 4*cep.ri*cep.vb*cep.d*cep.kt)^(1/2) - cep.kt^2) + cep.kt^2).^2 - cep.kt^4)./(4*cep.kt*cep.ri*cep.vb*cep.d);
u = -(cep.kt^4 - (2^(1/2)*(cep.kt*U*(cep.kt^3 - cep.kt*(cep.kt^4 + 4*cep.ri*cep.vb*cep.d*cep.kt)^(1/2) ...
    + 2*cep.ri*cep.vb*cep.d)).^(1/2) + cep.kt^2).^2)./(4*cep.kt*cep.ri*cep.vb*cep.d);

end

== matlab function indi_lib/Copter INDI Autotune/create diag ==
  data: u input; y output
function y = fcn(u)

y = diag(u);

== matlab function indi_lib/Incremental specific thrust/desired and measured specific thrust ==
  data: s_g_dt2 input; a_T_meas output; M_bg input; g input
function a_T_meas = fcn(s_g_dt2,M_bg, g)

a_b_meas = M_bg * s_g_dt2;

g_g = [0;0;g];
g_b = M_bg * g_g;
a_T_meas = a_b_meas(3) - g_b(3);

end
